simulink model "AEB_ClosedLoop_R2024a"  (R2024a)
settings: Solver=FixedStepDiscrete  StartTime=0.0  StopTime=15  FixedStep=aebDt  RelTol=1e-3
PreLoadFcn:
  | addpath(fileparts(get_param(bdroot,'FileName')));
model workspace (MAT data in the model file):
  aebDelay = 6
  aebDt = 0.02
  aebInitial = [0; 20; 46.5; 16; 0]
  aebLength = 4.5
  aebMemory = [0; 42; 4; 0; 1]
  aebNoise = [0 0.02 0.04 0.06 0.08 0.1 0.12 0.14 0.16 0.18 0.2 0.22 ... (3004 elements, 751x4)]
  aebObservation = [42; 4; 1]
  aebP = [0.02; 0.85; 8; 0.18; 3; 6; 4.5; 3; 0.12; 0.5; 1.7; 3; 6; 1; 0; 1.6; 20; 1.5]
  aebTs = 0.1
undefined symbols (not defined in the file or in its folder): aeb_sl_controller, aeb_sl_plant, aeb_sl_sensor
libraries: simulink x1
settings Model: Creator=Naceri  LastModifiedBy=Naceri
settings DataIOCC: SaveOutput=off  SignalLogging=off

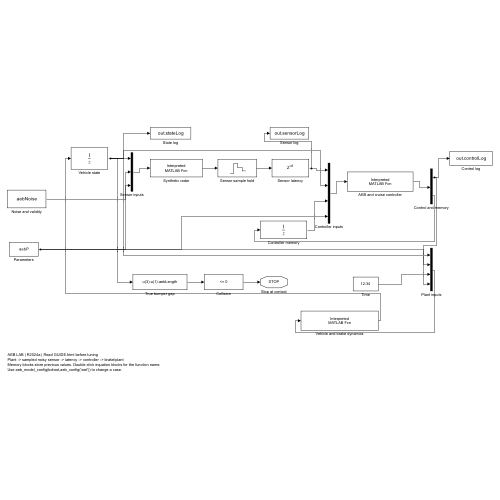
[thumbnail: Simulink's stored preview of the top-level diagram]
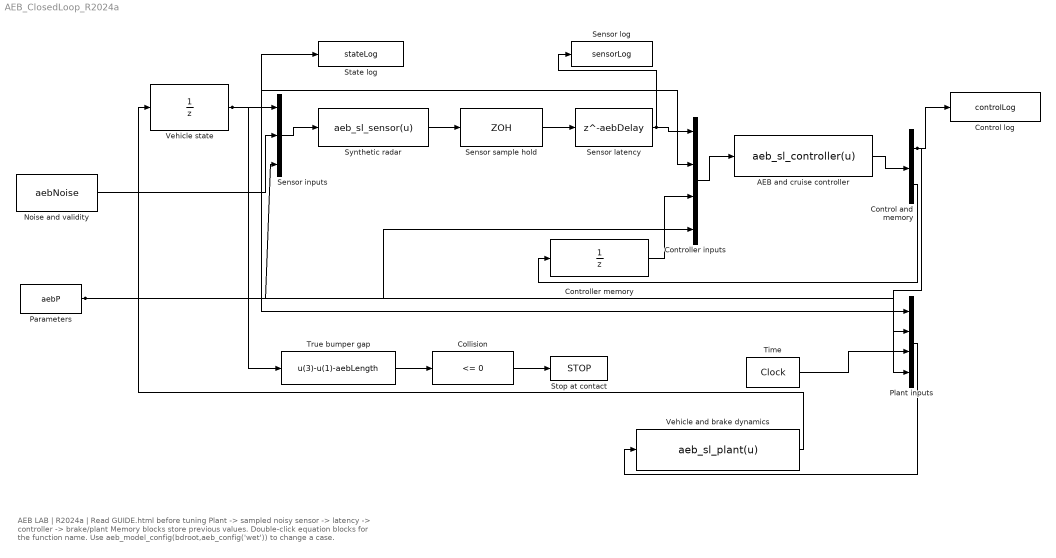
== system AEB_ClosedLoop_R2024a ==
  note: AEB LAB | R2024a | Read GUIDE.html before tuning
      | Plant -> sampled noisy sensor -> latency -> controller -> brake/plant
      | Memory blocks store previous values. Double-click equation blocks for the function name.
      | Use aeb_model_config(bdroot,aeb_config('wet')) to change a case.
  AEB and cruise controller : MATLABFcn  MATLABFcn=aeb_sl_controller(u)  OutputDimensions=10
  Collision : simulink/Logic and Bit Operations/Compare To Constant  relop=<=  const=0  OutDataTypeStr=boolean
  Control and memory : Demux  Outputs=[5 5]
  Control log : ToWorkspace  VariableName=controlLog  SaveFormat=Timeseries  SampleTime=-1
  Controller inputs : Mux
  Controller memory : UnitDelay  InitialCondition=aebMemory  SampleTime=aebDt  HasFrameUpgradeWarning=on
  Noise and validity : FromWorkspace  VariableName=aebNoise  SampleTime=aebDt  Interpolate=off  OutputAfterFinalValue=Holding final value
  Parameters : Constant  Value=aebP
  Plant inputs : Mux
  Sensor inputs : Mux  Inputs=3
  Sensor latency : Delay  DelayLength=aebDelay  InitialCondition=repmat(aebObservation,1,max(1,aebDelay))  SampleTime=aebDt
  Sensor log : ToWorkspace  VariableName=sensorLog  SaveFormat=Timeseries  SampleTime=-1
  Sensor sample hold : ZeroOrderHold  SampleTime=aebTs
  State log : ToWorkspace  VariableName=stateLog  SaveFormat=Timeseries  SampleTime=-1
  Stop at contact : Stop
  Synthetic radar : MATLABFcn  MATLABFcn=aeb_sl_sensor(u)  OutputDimensions=3
  Time : DigitalClock  SampleTime=aebDt
  True bumper gap : Fcn  Expr=u(3)-u(1)-aebLength
  Vehicle and brake dynamics : MATLABFcn  MATLABFcn=aeb_sl_plant(u)  OutputDimensions=5
  Vehicle state : UnitDelay  InitialCondition=aebInitial  SampleTime=aebDt  HasFrameUpgradeWarning=on
  wires:
  Vehicle and brake dynamics/1 -> Vehicle state/1
  Vehicle state/1 -> Sensor inputs/1, Controller inputs/2, Plant inputs/1, State log/1, True bumper gap/1
  Noise and validity/1 -> Sensor inputs/2
  Parameters/1 -> Sensor inputs/3, Controller inputs/4, Plant inputs/4
  Sensor inputs/1 -> Synthetic radar/1
  Synthetic radar/1 -> Sensor sample hold/1
  Sensor sample hold/1 -> Sensor latency/1
  Sensor latency/1 -> Controller inputs/1, Sensor log/1
  Controller memory/1 -> Controller inputs/3
  Controller inputs/1 -> AEB and cruise controller/1
  AEB and cruise controller/1 -> Control and memory/1
  Control and memory/2 -> Controller memory/1
  Control and memory/1 -> Plant inputs/2, Control log/1
  Time/1 -> Plant inputs/3
  Plant inputs/1 -> Vehicle and brake dynamics/1
  True bumper gap/1 -> Collision/1
  Collision/1 -> Stop at contact/1
